simulink model "testing"  (R2025b)
settings: Solver=VariableStepAuto  StartTime=0.0  StopTime=50  RelTol=1e-3
values from neighbouring files (symbols this model uses):
  Area = 2*L*Width    (= 0.072)    [quad_params.m]
  end_h = 0.03    [quad_params.m]
  g = 9.81    [quad_params.m]
  h = [0 ... (first row only)    [Madgwick.m]    (also in quad_params.m = 0.2; umich_learning.m = x(:,1))
  h0 = Ts    (= 0.001)    [quad_params.m]
  inertia_mx = [Ixx; Iyy; Izz;]    [quad_params.m]
  init_h = 0.03    [quad_params.m]
  K_alloc = Alloc \ diag([W, 1, 1, 1])    [quad_params.m]
  r0_angle = 1000    [quad_params.m]
  r0_position = 1    [quad_params.m]
  rho_air = 1.225    [quad_params.m]
  rho_water = 1000    [quad_params.m]
  Trot = 0.01    [quad_params.m]
  Ts = 0.001    [get_noise.m]    (also in quad_params.m; test.m = 0.002)
  W = 0.7 + 4*m_prop    (= 0.74)    [quad_params.m]
undefined symbols (not defined in the file or in its folder): Alloc_2, b0, b0_pitch, b0_roll, b0_x, b0_y, b0_yaw, b0_z, beta1_pitch, beta1_roll, beta1_x, beta1_y, beta1_yaw, beta1_z, beta2_pitch, beta2_roll, beta2_x, beta2_y, beta2_yaw, beta2_z, beta3_pitch, beta3_roll, beta3_x, beta3_y, beta3_yaw, beta3_z, m, wc, wc_pitch, wc_roll, wc_x, wc_y, wc_yaw, wc_z, wo
libraries: simulink x3, shareduavrstlib x2, SignalEditorBlockLib x2, aerolibwind2 x1
(part 2 of 2)

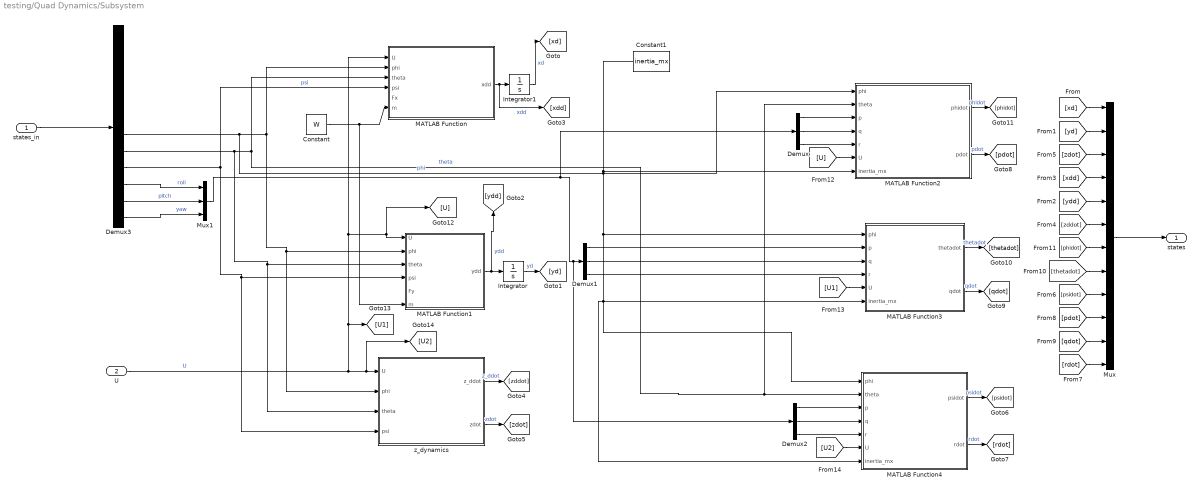
== system testing/Quad Dynamics/Subsystem ==
  states_in : Inport
  U : Inport  Port=2
  Constant : Constant  Value=W
  Constant1 : Constant  Value=inertia_mx
  Demux : Demux  Outputs=3
  Demux1 : Demux  Outputs=3
  Demux2 : Demux  Outputs=3
  Demux3 : Demux  Outputs=12
  Integrator : Integrator
  Integrator1 : Integrator
  MATLAB Function : MATLAB Function  TreatAsAtomicUnit=on
  MATLAB Function1 : MATLAB Function  TreatAsAtomicUnit=on
  MATLAB Function2 : MATLAB Function  TreatAsAtomicUnit=on
  MATLAB Function3 : MATLAB Function  TreatAsAtomicUnit=on
  MATLAB Function4 : MATLAB Function  TreatAsAtomicUnit=on
  Mux : Mux  Inputs=12
  Mux1 : Mux  Inputs=3
  z_dynamics : Subsystem
  states : Outport
  wires:
  MATLAB Function/1(xdd) -> [xdd], Integrator1/1  "xdd"
  MATLAB Function1/1(ydd) -> [ydd], Integrator/1  "ydd"
  Mux/1 -> states/1
  states_in/1 -> Demux3/1
  U/1 -> [U2], z_dynamics/1(U), MATLAB Function/1(U), [U], MATLAB Function1/1(U), [U1]  "U"
  Demux3/7 -> MATLAB Function3/1(phi), MATLAB Function4/1(phi), MATLAB Function2/1(phi), MATLAB Function/2(phi), z_dynamics/2(phi), MATLAB Function1/2(phi)  "phi"
  Demux3/8 -> z_dynamics/3(theta), MATLAB Function1/3(theta), MATLAB Function2/2(theta), MATLAB Function4/2(theta), MATLAB Function/3(theta)  "theta"
  Demux3/9 -> z_dynamics/4(psi), MATLAB Function1/4(psi), MATLAB Function/4(psi)  "psi"
  Constant/1 -> MATLAB Function/6(m), MATLAB Function1/6(m)
  Constant1/1 -> MATLAB Function4/7(inertia_mx), MATLAB Function3/6(inertia_mx), MATLAB Function2/7(inertia_mx)
  Demux3/11 -> Mux1/2  "pitch"
  Demux3/12 -> Mux1/3  "yaw"
  Demux3/10 -> Mux1/1  "roll"
  Mux1/1 -> Demux/1, Demux2/1, Demux1/1
  Demux1/1 -> MATLAB Function3/2(p)
  Demux1/2 -> MATLAB Function3/3(q)
  Demux1/3 -> MATLAB Function3/4(r)
  Demux2/1 -> MATLAB Function4/3(p)
  Demux2/2 -> MATLAB Function4/4(q)
  Demux2/3 -> MATLAB Function4/5(r)
  Demux/1 -> MATLAB Function2/3(p)
  Demux/2 -> MATLAB Function2/4(q)
  Demux/3 -> MATLAB Function2/5(r)
  Integrator1/1 -> [xd]  "xd"
  [xd] -> Mux/1
  Integrator/1 -> [yd]  "yd"
  [yd] -> Mux/2
  [ydd] -> Mux/5
  [xdd] -> Mux/4
  z_dynamics/1(z_ddot) -> [zddot]  "z_ddot"
  [zddot] -> Mux/6
  z_dynamics/2(zdot) -> [zdot]  "zdot"
  [zdot] -> Mux/3
  MATLAB Function4/1(psidot) -> [psidot]  "psidot"
  [psidot] -> Mux/9
  MATLAB Function4/2(rdot) -> [rdot]  "rdot"
  [rdot] -> Mux/12
  MATLAB Function2/2(pdot) -> [pdot]  "pdot"
  [pdot] -> Mux/10
  MATLAB Function3/2(qdot) -> [qdot]  "qdot"
  [qdot] -> Mux/11
  MATLAB Function3/1(thetadot) -> [thetadot]  "thetadot"
  [thetadot] -> Mux/8
  MATLAB Function2/1(phidot) -> [phidot]  "phidot"
  [phidot] -> Mux/7
  [U] -> MATLAB Function2/6(U)
  [U1] -> MATLAB Function3/5(U)
  [U2] -> MATLAB Function4/6(U)

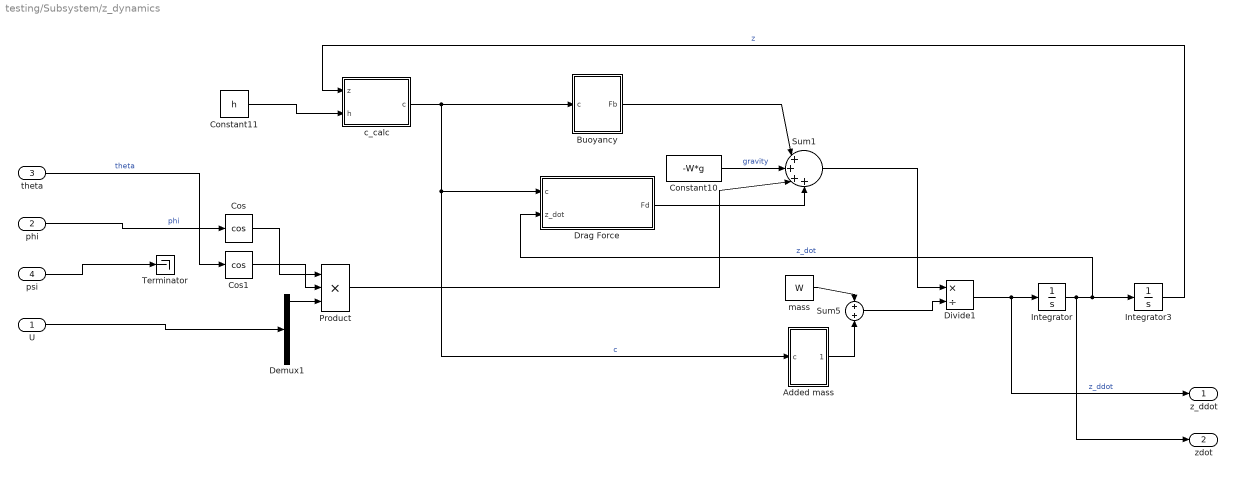
== system testing/Subsystem/z_dynamics ==
  U : Inport
  phi : Inport  Port=2
  theta : Inport  Port=3
  psi : Inport  Port=4
  Added mass : Subsystem
  Buoyancy : Subsystem
  Constant10 : Constant  Value=-W*g
  Constant11 : Constant  Value=h
  Cos : Trigonometry  Operator=cos
  Cos1 : Trigonometry  Operator=cos
  Demux1 : Demux
  Divide1 : Product  Inputs=*/
  Drag Force : Subsystem
  Integrator : Integrator
  Integrator3 : Integrator  InitialCondition=init_h
  Product : Product  Inputs=3
  Sum1 : Sum  Inputs=|++++
  Sum5 : Sum
  Terminator : Terminator
  c_calc : MATLAB Function  TreatAsAtomicUnit=on
  mass : Constant  Value=W
  z_ddot : Outport
  zdot : Outport  Port=2
  wires:
  phi/1 -> Cos/1  "phi"
  theta/1 -> Cos1/1  "theta"
  Cos/1 -> Product/1
  Cos1/1 -> Product/2
  Demux1/1 -> Product/3
  psi/1 -> Terminator/1
  Sum1/1 -> Divide1/1
  c_calc/1(c) -> Buoyancy/1(c), Added mass/1(c), Drag Force/1(c)  "c"
  Product/1 -> Sum1/3
  Added mass/1(m_a) -> Sum5/2
  mass/1 -> Sum5/1
  Sum5/1 -> Divide1/2
  Integrator3/1 -> c_calc/1(z)  "z"
  Integrator/1 -> Drag Force/2(z_dot), Integrator3/1, zdot/1  "z_dot"
  Drag Force/1(Fd) -> Sum1/4
  Divide1/1 -> z_ddot/1, Integrator/1  "z_ddot"
  Buoyancy/1(Fb) -> Sum1/1
  Constant10/1 -> Sum1/2  "gravity"
  Constant11/1 -> c_calc/2(h)
  U/1 -> Demux1/1

== system testing/Subsystem3/Added mass ==
  c : Inport
  Product1 : Product
  added_mass : Constant  Value=0.005*rho_water
  m_a : Outport
  wires:
  added_mass/1 -> Product1/1
  Product1/1 -> m_a/1
  c/1 -> Product1/2

== system testing/Subsystem3/Buoyancy ==
  c : Inport
  Constant1 : Constant  Value=rho_water*Area*g
  Product : Product
  Fb : Outport
  wires:
  Constant1/1 -> Product/2
  c/1 -> Product/1
  Product/1 -> Fb/1  "buoyancy"

== system testing/Subsystem3/Drag Force ==
  c : Inport
  z_dot : Inport  Port=2
  Abs : Abs  SaturateOnIntegerOverflow=off
  Constant : Constant  Value=h
  Constant10 : Constant
  Constant11 : Constant  Value=Area
  Constant7 : Constant  Value=rho_air
  Constant8 : Constant  Value=rho_water
  Constant9 : Constant  Value=-0.5
  Divide : Product  Inputs=*/
  Product3 : Product
  Product4 : Product
  Product5 : Product  Inputs=5
  Sum2 : Sum
  Sum3 : Sum  Inputs=+-
  Fd : Outport
  wires:
  Divide/1 -> Sum3/2, Product4/2
  Product5/1 -> Fd/1  "drag force"
  Product4/1 -> Sum2/2  "water drag"
  Constant11/1 -> Product5/5
  Sum3/1 -> Product3/2
  Constant8/1 -> Product4/1  "water"
  Constant10/1 -> Sum3/1
  Sum2/1 -> Product5/1
  Constant9/1 -> Product5/2
  z_dot/1 -> Abs/1, Product5/3
  Abs/1 -> Product5/4
  Product3/1 -> Sum2/1  "air drag"
  Constant7/1 -> Product3/1  "air"
  c/1 -> Divide/1
  Constant/1 -> Divide/2

== system testing/plant/Added mass ==
  c : Inport
  Product1 : Product
  added_mass : Constant  Value=0.005*rho_water
  m_a : Outport
  wires:
  c/1 -> Product1/2
  Product1/1 -> m_a/1
  added_mass/1 -> Product1/1

== system testing/plant/Buoyancy ==
  c : Inport
  Constant1 : Constant  Value=rho_water*Area*g
  Product : Product
  Fb : Outport
  wires:
  Product/1 -> Fb/1  "buoyancy"
  c/1 -> Product/1
  Constant1/1 -> Product/2

== system testing/plant/Drag Force ==
  c : Inport
  z_dot : Inport  Port=2
  Abs : Abs  SaturateOnIntegerOverflow=off
  Constant : Constant  Value=h
  Constant10 : Constant
  Constant11 : Constant  Value=Area
  Constant7 : Constant  Value=rho_air
  Constant8 : Constant  Value=rho_water
  Constant9 : Constant  Value=-0.5
  Divide : Product  Inputs=*/
  Product3 : Product
  Product4 : Product
  Product5 : Product  Inputs=5
  Sum2 : Sum
  Sum3 : Sum  Inputs=+-
  Fd : Outport
  wires:
  Constant/1 -> Divide/2
  c/1 -> Divide/1
  Constant7/1 -> Product3/1  "air"
  Product3/1 -> Sum2/1  "air drag"
  Abs/1 -> Product5/4
  z_dot/1 -> Product5/3, Abs/1
  Constant9/1 -> Product5/2
  Sum2/1 -> Product5/1
  Constant10/1 -> Sum3/1
  Constant8/1 -> Product4/1  "water"
  Sum3/1 -> Product3/2
  Constant11/1 -> Product5/5
  Product4/1 -> Sum2/2  "water drag"
  Product5/1 -> Fd/1  "drag force"
  Divide/1 -> Product4/2, Sum3/2

== system testing/ref_z/Min Jerk Trajectory1 ==
  Constant1 : Constant  Value="[0    5    10   15   20   25]"
  Minimum Jerk Polynomial Trajectory : shareduavrstlib/Minimum Jerk Polynomial Trajectory  ShowBCInputPort=off  ShowPolynomialCoefs=off  ShowStatusOutputPort=off  TimeAllocation=off  TimeWeight=100  MinSegmentTime=0.1  MaxSegmentTime=1  MaxIteration=1500  MaxTime=10  SimulateUsing=Interpreted execution
  Ramp : simulink/Sources/Ramp  slope=1  start=0  InitialOutput=0
  Selector : Selector  InputPortWidth=2  IndexOptions=Index vector (dialog)  Indices=1  OutputSizes=1
  Selector1 : Selector  InputPortWidth=2  IndexOptions=Index vector (dialog)  Indices=1  OutputSizes=1
  Terminator : Terminator
  Terminator1 : Terminator
  Terminator2 : Terminator
  Waypoints2 : Constant  Value="[init_h  init_h  2.0  3.0  2.0  end_h;0 0 0 0 0 0];"
  ref : Outport
  dref : Outport  Port=2
  wires:
  Minimum Jerk Polynomial Trajectory/3 -> Terminator/1
  Waypoints2/1 -> Minimum Jerk Polynomial Trajectory/2
  Ramp/1 -> Minimum Jerk Polynomial Trajectory/1
  Selector1/1 -> dref/1  "ref"
  Constant1/1 -> Minimum Jerk Polynomial Trajectory/3
  Minimum Jerk Polynomial Trajectory/2 -> Selector1/1
  Minimum Jerk Polynomial Trajectory/1 -> Selector/1  "height"
  Selector/1 -> ref/1  "ref"
  Minimum Jerk Polynomial Trajectory/4 -> Terminator1/1
  Minimum Jerk Polynomial Trajectory/5 -> Terminator2/1

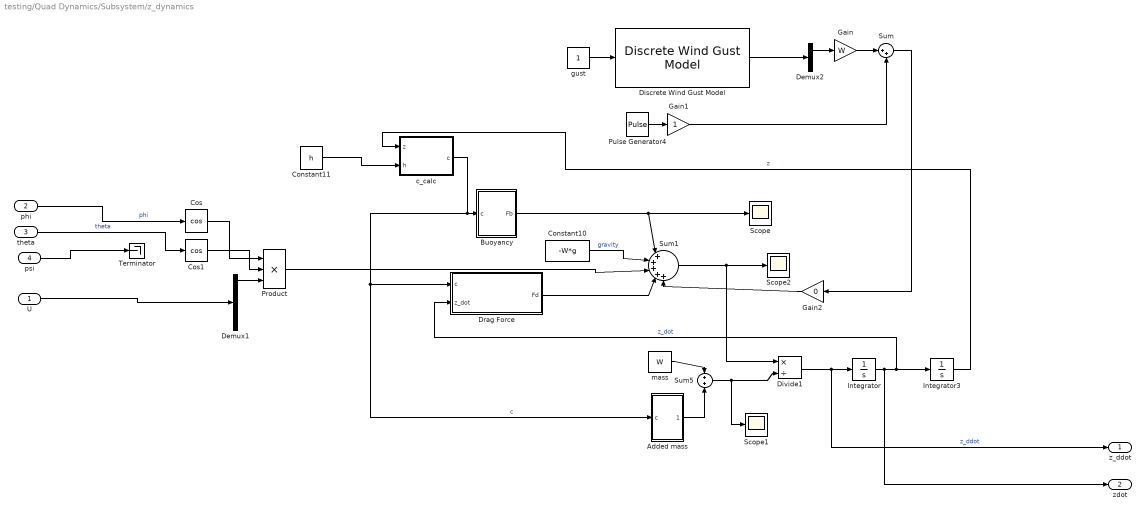
== system testing/Quad Dynamics/Subsystem/z_dynamics ==
  U : Inport
  phi : Inport  Port=2
  theta : Inport  Port=3
  psi : Inport  Port=4
  Added mass : Subsystem
  Buoyancy : Subsystem
  Constant10 : Constant  Value=-W*g
  Constant11 : Constant  Value=h
  Cos : Trigonometry  Operator=cos
  Cos1 : Trigonometry  Operator=cos
  Demux1 : Demux
  Demux2 : Demux  Outputs=3
  Discrete Wind Gust Model : aerolibwind2/Discrete Wind Gust Model  units=Metric (MKS)  Gx=on  Gy=off  Gz=off  t_0=7  d_m=[1 0.5 0.5]  v_m=[2 2 2]
  Divide1 : Product  Inputs=*/
  Drag Force : Subsystem
  Gain : Gain  Gain=W
  Gain1 : Gain
  Gain2 : Gain  Gain=0
  Integrator : Integrator
  Integrator3 : Integrator  InitialCondition=init_h
  Product : Product  Inputs=3
  Pulse Generator4 : DiscretePulseGenerator  PulseType=Time based  Amplitude=5  Period=5  PulseWidth=30  PhaseDelay=5
  Scope : Scope
      settings: ActiveDisplayYMinimum=3.324205069659222  ActiveDisplayYMaximum=24.046643881148977  DataLoggingVariableName=ScopeData4
  Scope1 : Scope
      settings: ActiveDisplayYMinimum=1.2962500000000001  ActiveDisplayYMaximum=1.7337500000000001  DataLoggingVariableName=ScopeData8
  Scope2 : Scope
      settings: ActiveDisplayYMinimum=-2.7468  ActiveDisplayYMaximum=24.721200000000003  DataLoggingVariableName=ScopeData10
  Sum : Sum  Inputs=|++
  Sum1 : Sum  Inputs=|+++++
  Sum5 : Sum
  Terminator : Terminator
  c_calc : MATLAB Function  TreatAsAtomicUnit=on
  gust : Constant
  mass : Constant  Value=W
  z_ddot : Outport
  zdot : Outport  Port=2
  wires:
  phi/1 -> Cos/1  "phi"
  theta/1 -> Cos1/1  "theta"
  Cos/1 -> Product/1
  Cos1/1 -> Product/2
  Demux1/1 -> Product/3
  psi/1 -> Terminator/1
  Sum1/1 -> Scope2/1, Divide1/1
  c_calc/1(c) -> Added mass/1(c), Drag Force/1(c), Buoyancy/1(c)  "c"
  Product/1 -> Sum1/3
  Added mass/1(m_a) -> Sum5/2
  mass/1 -> Sum5/1
  Sum5/1 -> Scope1/1, Divide1/2
  Integrator3/1 -> c_calc/1(z)  "z"
  Integrator/1 -> Drag Force/2(z_dot), Integrator3/1, zdot/1  "z_dot"
  Drag Force/1(Fd) -> Sum1/4
  Divide1/1 -> z_ddot/1, Integrator/1  "z_ddot"
  Buoyancy/1(Fb) -> Sum1/1, Scope/1
  Constant10/1 -> Sum1/2  "gravity"
  Constant11/1 -> c_calc/2(h)
  U/1 -> Demux1/1
  Gain1/1 -> Sum/2
  Discrete Wind Gust Model/1 -> Demux2/1
  Demux2/1 -> Gain/1
  Gain/1 -> Sum/1
  Pulse Generator4/1 -> Gain1/1
  Sum/1 -> Gain2/1
  gust/1 -> Discrete Wind Gust Model/1
  Gain2/1 -> Sum1/5

== system testing/Subsystem/z_dynamics/Added mass ==
  c : Inport
  Product1 : Product
  added_mass : Constant  Value=0.005*rho_water
  m_a : Outport
  wires:
  added_mass/1 -> Product1/1
  Product1/1 -> m_a/1
  c/1 -> Product1/2

== system testing/Subsystem/z_dynamics/Buoyancy ==
  c : Inport
  Constant1 : Constant  Value=rho_water*Area*g
  Product : Product
  Fb : Outport
  wires:
  Constant1/1 -> Product/2
  c/1 -> Product/1
  Product/1 -> Fb/1  "buoyancy"

== system testing/Subsystem/z_dynamics/Drag Force ==
  c : Inport
  z_dot : Inport  Port=2
  Abs : Abs  SaturateOnIntegerOverflow=off
  Constant : Constant  Value=h
  Constant10 : Constant
  Constant11 : Constant  Value=Area
  Constant7 : Constant  Value=rho_air
  Constant8 : Constant  Value=rho_water
  Constant9 : Constant  Value=-0.5
  Divide : Product  Inputs=*/
  Product3 : Product
  Product4 : Product
  Product5 : Product  Inputs=5
  Sum2 : Sum
  Sum3 : Sum  Inputs=+-
  Fd : Outport
  wires:
  Divide/1 -> Sum3/2, Product4/2
  Product5/1 -> Fd/1  "drag force"
  Product4/1 -> Sum2/2  "water drag"
  Constant11/1 -> Product5/5
  Sum3/1 -> Product3/2
  Constant8/1 -> Product4/1  "water"
  Constant10/1 -> Sum3/1
  Sum2/1 -> Product5/1
  Constant9/1 -> Product5/2
  z_dot/1 -> Abs/1, Product5/3
  Abs/1 -> Product5/4
  Product3/1 -> Sum2/1  "air drag"
  Constant7/1 -> Product3/1  "air"
  c/1 -> Divide/1
  Constant/1 -> Divide/2

== system testing/Quad Dynamics/Subsystem/z_dynamics/Added mass ==
  c : Inport
  Product1 : Product
  added_mass : Constant  Value=0.005*rho_water
  m_a : Outport
  wires:
  added_mass/1 -> Product1/1
  Product1/1 -> m_a/1
  c/1 -> Product1/2

== system testing/Quad Dynamics/Subsystem/z_dynamics/Buoyancy ==
  c : Inport
  Constant1 : Constant  Value=rho_water*Area*g
  Product : Product
  Fb : Outport
  wires:
  Constant1/1 -> Product/2
  c/1 -> Product/1
  Product/1 -> Fb/1  "buoyancy"

== system testing/Quad Dynamics/Subsystem/z_dynamics/Drag Force ==
  c : Inport
  z_dot : Inport  Port=2
  Abs : Abs  SaturateOnIntegerOverflow=off
  Constant : Constant  Value=h
  Constant10 : Constant
  Constant11 : Constant  Value=Area
  Constant7 : Constant  Value=rho_air
  Constant8 : Constant  Value=rho_water
  Constant9 : Constant  Value=-0.5
  Divide : Product  Inputs=*/
  Product3 : Product
  Product4 : Product
  Product5 : Product  Inputs=5
  Sum2 : Sum
  Sum3 : Sum  Inputs=+-
  Fd : Outport
  wires:
  Divide/1 -> Sum3/2, Product4/2
  Product5/1 -> Fd/1  "drag force"
  Product4/1 -> Sum2/2  "water drag"
  Constant11/1 -> Product5/5
  Sum3/1 -> Product3/2
  Constant8/1 -> Product4/1  "water"
  Constant10/1 -> Sum3/1
  Sum2/1 -> Product5/1
  Constant9/1 -> Product5/2
  z_dot/1 -> Abs/1, Product5/3
  Abs/1 -> Product5/4
  Product3/1 -> Sum2/1  "air drag"
  Constant7/1 -> Product3/1  "air"
  c/1 -> Divide/1
  Constant/1 -> Divide/2

== matlab function testing/ADRC_pitch/TD1/fhan ==
  data: e input; u output; v2 input; r0 input; h0 input

function u = fhan(e, v2, r0, h0)

d = r0*h0^2;
a0 = h0*v2;
y = e + a0;

a1 = sqrt(d*(d + 8*abs(y)));
a2 = a0 + sign(y)*(a1 - d)/2;

sy = (sign(y + d) - sign(y - d))/2;
a = (a0 + y - a2)*sy + a2;

sa = (sign(a + d) - sign(a - d))/2;

u = -r0*(a/d - sign(a))*sa - r0*sign(a);

end

== matlab function testing/ADRC_roll/TD1/fhan ==
  data: e input; u output; v2 input; r0 input; h0 input

function u = fhan(e, v2, r0, h0)

d = r0*h0^2;
a0 = h0*v2;
y = e + a0;

a1 = sqrt(d*(d + 8*abs(y)));
a2 = a0 + sign(y)*(a1 - d)/2;

sy = (sign(y + d) - sign(y - d))/2;
a = (a0 + y - a2)*sy + a2;

sa = (sign(a + d) - sign(a - d))/2;

u = -r0*(a/d - sign(a))*sa - r0*sign(a);

end

== matlab function testing/ADRC_x/TD1/fhan ==
  data: e input; u output; v2 input; r0 input; h0 input

function u = fhan(e, v2, r0, h0)

d = r0*h0^2;
a0 = h0*v2;
y = e + a0;

a1 = sqrt(d*(d + 8*abs(y)));
a2 = a0 + sign(y)*(a1 - d)/2;

sy = (sign(y + d) - sign(y - d))/2;
a = (a0 + y - a2)*sy + a2;

sa = (sign(a + d) - sign(a - d))/2;

u = -r0*(a/d - sign(a))*sa - r0*sign(a);

end

== matlab function testing/ADRC_y/TD1/fhan ==
  data: e input; u output; v2 input; r0 input; h0 input

function u = fhan(e, v2, r0, h0)

d = r0*h0^2;
a0 = h0*v2;
y = e + a0;

a1 = sqrt(d*(d + 8*abs(y)));
a2 = a0 + sign(y)*(a1 - d)/2;

sy = (sign(y + d) - sign(y - d))/2;
a = (a0 + y - a2)*sy + a2;

sa = (sign(a + d) - sign(a - d))/2;

u = -r0*(a/d - sign(a))*sa - r0*sign(a);

end

== matlab function testing/ADRC_yaw/TD1/fhan ==
  data: e input; u output; v2 input; r0 input; h0 input

function u = fhan(e, v2, r0, h0)

d = r0*h0^2;
a0 = h0*v2;
y = e + a0;

a1 = sqrt(d*(d + 8*abs(y)));
a2 = a0 + sign(y)*(a1 - d)/2;

sy = (sign(y + d) - sign(y - d))/2;
a = (a0 + y - a2)*sy + a2;

sa = (sign(a + d) - sign(a - d))/2;

u = -r0*(a/d - sign(a))*sa - r0*sign(a);

end

== matlab function testing/LADRC/MATLAB Function ==
  data: z input; y output; e input
function y = fcn(z, e)

thresh_h = 0.1;

if z<thresh_h
    y = 0;
else
    y = e;
end

== matlab function testing/ADRC_z/TD1/fhan ==
  data: e input; u output; v2 input; r0 input; h0 input

function u = fhan(e, v2, r0, h0)

d = r0*h0^2;
a0 = h0*v2;
y = e + a0;

a1 = sqrt(d*(d + 8*abs(y)));
a2 = a0 + sign(y)*(a1 - d)/2;

sy = (sign(y + d) - sign(y - d))/2;
a = (a0 + y - a2)*sy + a2;

sa = (sign(a + d) - sign(a - d))/2;

u = -r0*(a/d - sign(a))*sa - r0*sign(a);

end

== matlab function testing/Quad Dynamics/Subsystem/MATLAB Function ==
  data: U input; phi input; xdd output; theta input; psi input; Fx input; m input
function xdd = x_dynamics(U, phi, theta, psi, Fx, m)

T = U(1);
xdd = (T/m)*(cos(psi)*sin(theta)*cos(phi) ...
               + sin(psi)*sin(phi)) + Fx/m;

end

== matlab function testing/Quad Dynamics/Subsystem/MATLAB Function1 ==
  data: U input; ydd output; phi input; theta input; psi input; Fy input; m input
function ydd = y_dynamics(U, phi, theta, psi, Fy, m)

T = U(1);

ydd = (T/m)*(sin(psi)*sin(theta)*cos(phi) ...
               - cos(psi)*sin(phi)) + Fy/m;

end

== matlab function testing/Quad Dynamics/Subsystem/MATLAB Function2 ==
  data: phi input size=1; phidot output size=1; theta input size=1; p input size=1; q input size=1; r input size=1; U input; inertia_mx input; pdot output size=1
function [phidot, pdot] = roll_dynamics( ...
    phi, theta, p, q, r, U, inertia_mx)

Ix = inertia_mx(1);
Iy = inertia_mx(2);
Iz = inertia_mx(3);

tau_roll = U(2);

phidot = p + sin(phi)*tan(theta)*q ...
           + cos(phi)*tan(theta)*r;

pdot = (tau_roll + (Iy-Iz)*q*r)/Ix;

end

== matlab function testing/Quad Dynamics/Subsystem/MATLAB Function3 ==
  data: phi input size=1; thetadot output size=1; p input size=1; q input size=1; r input size=1; U input size=[4 1]; inertia_mx input size=[3 1]; qdot output size=1
function [thetadot, qdot] = pitch_dynamics( ...
    phi, p, q, r, U, inertia_mx)

Ix = inertia_mx(1);
Iy = inertia_mx(2);
Iz = inertia_mx(3);

tau_pitch = U(3);

thetadot = cos(phi)*q - sin(phi)*r;

qdot = (tau_pitch + (Iz-Ix)*p*r)/Iy;

end

== matlab function testing/Quad Dynamics/Subsystem/MATLAB Function4 ==
  data: phi input size=1; psidot output size=1; theta input size=1; p input size=1; q input size=1; r input size=1; U input; inertia_mx input; rdot output size=1
function [psidot, rdot] = yaw_dynamics( ...
    phi, theta, p, q, r, U, inertia_mx)

Ix = inertia_mx(1);
Iy = inertia_mx(2);
Iz = inertia_mx(3);

psidot = 0;
rdot = 0;

tau_yaw = U(4);

psidot = (sin(phi)*q + cos(phi)*r)/cos(theta);

rdot = (tau_yaw + (Ix-Iy)*p*q)/Iz;

end

== matlab function testing/Quad Dynamics/Subsystem/z_dynamics/c_calc ==
  data: z input; c output; h input
function c = fcn(z, h)

if z > h/2
    c = 0;
elseif z < -h/2
    c = h;
else 
    c = h/2 - z;
end

== matlab function testing/Subsystem3/c_calc ==
  data: z input; c output; h input
function c = fcn(z, h)

if z > h/2
    c = 0;
elseif z < -h/2
    c = h;
else 
    c = h/2 - z;
end

== matlab function testing/plant/c_calc ==
  data: z input; c output; h input
function c = fcn(z, h)

if z > h/2
    c = 0;
elseif z < -h/2
    c = h;
else 
    c = h/2 - z;
end

== matlab function testing/Subsystem/MATLAB Function ==
  data: U input; phi input; xdd output; theta input; psi input; Fx input; m input
function xdd = x_dynamics(U, phi, theta, psi, Fx, m)

T = U(1);
xdd = (T/m)*(cos(psi)*sin(theta)*cos(phi) ...
               + sin(psi)*sin(phi)) + Fx/m;

end

== matlab function testing/Subsystem/MATLAB Function1 ==
  data: U input; ydd output; phi input; theta input; psi input; Fy input; m input
function ydd = y_dynamics(U, phi, theta, psi, Fy, m)

T = U(1);

ydd = (T/m)*(sin(psi)*sin(theta)*cos(phi) ...
               - cos(psi)*sin(phi)) + Fy/m;

end

== matlab function testing/Subsystem/z_dynamics/c_calc ==
  data: z input; c output; h input
function c = fcn(z, h)

if z > h/2
    c = 0;
elseif z < -h/2
    c = h;
else 
    c = h/2 - z;
end

== matlab function testing/Subsystem/MATLAB Function2 ==
  data: phi input; phidot output; theta input; p input; q input; r input; U input; inertia_mx input; pdot output
function [phidot, pdot] = roll_dynamics( ...
    phi, theta, p, q, r, U, inertia_mx)

Ix = inertia_mx(1);
Iy = inertia_mx(2);
Iz = inertia_mx(3);

tau_roll = U(2);


phidot = p + sin(phi)*tan(theta)*q ...
           + cos(phi)*tan(theta)*r;

pdot = (tau_roll + (Iy-Iz)*q*r)/Ix;

end

== matlab function testing/Subsystem/MATLAB Function3 ==
  data: phi input; thetadot output; p input; q input; r input; U input; inertia_mx input; qdot output
function [thetadot, qdot] = pitch_dynamics( ...
    phi, p, q, r, U, inertia_mx)

Ix = inertia_mx(1);
Iy = inertia_mx(2);
Iz = inertia_mx(3);

tau_pitch = U(3);

thetadot = cos(phi)*q - sin(phi)*r;

qdot = (tau_pitch + (Iz-Ix)*p*r)/Iy;

end

== matlab function testing/Subsystem/MATLAB Function4 ==
  data: phi input; psidot output; theta input; p input; q input; r input; U input; inertia_mx input; rdot output
function [psidot, rdot] = yaw_dynamics( ...
    phi, theta, p, q, r, U, inertia_mx)

Ix = inertia_mx(1);
Iy = inertia_mx(2);
Iz = inertia_mx(3);


tau_yaw = U(4);

psidot = (sin(phi)*q + cos(phi)*r)/cos(theta);

rdot = (tau_yaw + (Ix-Iy)*p*q)/Iz;

end
